simulink model "TP10_Examen_essuie_glaces_automatiques_simulink"  (R2022b)
settings: Solver=VariableStepAuto  StartTime=0.0  StopTime=inf  RelTol=1e-3
libraries: simulink x12
settings Model: Creator=HP  LastModifiedBy=HP

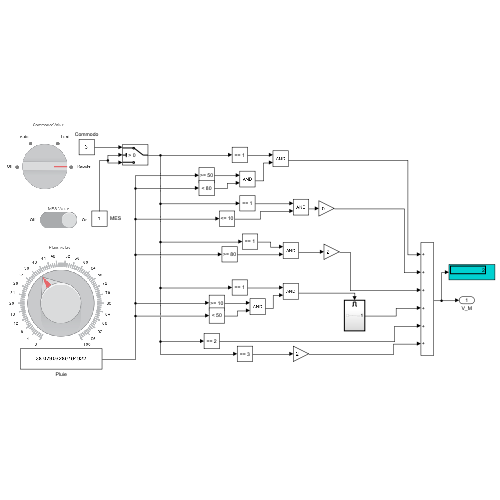
[thumbnail: Simulink's stored preview of the top-level diagram]
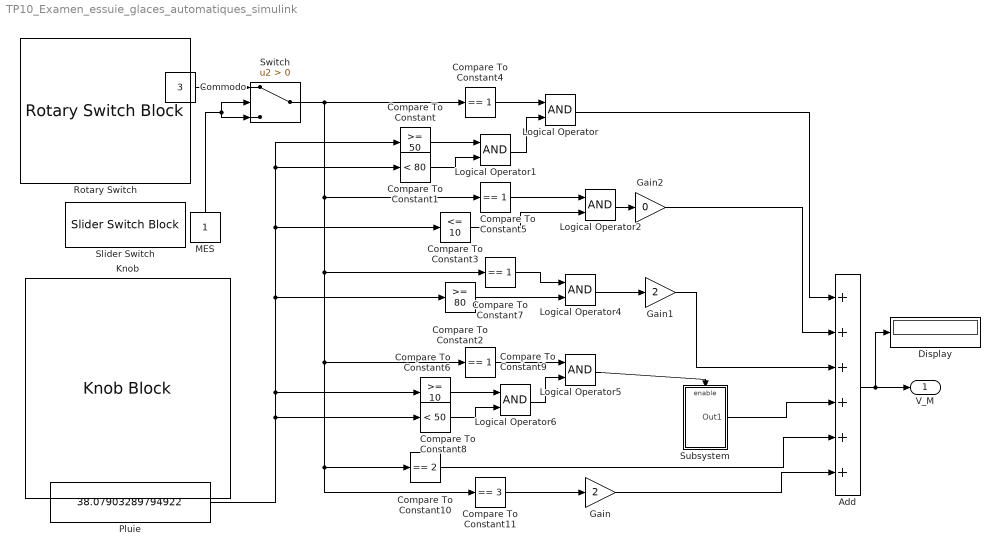
== system TP10_Examen_essuie_glaces_automatiques_simulink ==
  Add : Sum  Inputs=6
  Commodo : Constant  Value=3
  Compare To Constant : simulink/Logic and Bit Operations/Compare To Constant  relop=>=  const=50  OutDataTypeStr=boolean
  Compare To Constant1 : simulink/Logic and Bit Operations/Compare To Constant  relop=<  const=80  OutDataTypeStr=boolean
  Compare To Constant10 : simulink/Logic and Bit Operations/Compare To Constant  relop===  const=2  OutDataTypeStr=boolean
  Compare To Constant11 : simulink/Logic and Bit Operations/Compare To Constant  relop===  const=3  OutDataTypeStr=boolean
  Compare To Constant2 : simulink/Logic and Bit Operations/Compare To Constant  relop=>=  const=80  OutDataTypeStr=boolean
  Compare To Constant3 : simulink/Logic and Bit Operations/Compare To Constant  relop=<=  const=10  OutDataTypeStr=boolean
  Compare To Constant{4..5,7,9} (4 alike) : simulink/Logic and Bit Operations/Compare To Constant  relop===  const=1  OutDataTypeStr=boolean
  Compare To Constant6 : simulink/Logic and Bit Operations/Compare To Constant  relop=>=  const=10  OutDataTypeStr=boolean
  Compare To Constant8 : simulink/Logic and Bit Operations/Compare To Constant  relop=<  const=50  OutDataTypeStr=boolean
  Display : Display
  Gain : Gain  Gain=2
  Gain1 : Gain  Gain=2
  Gain2 : Gain  Gain=0
  Knob : KnobBlock
  Logical Operator{,1..2,4..6} (6 alike) : Logic  AllPortsSameDT=off  OutDataTypeStr=boolean
  MES : Constant
  Pluie : Constant  Value=38.07903289794922
  Rotary Switch : RotarySwitchBlock
      settings: Values={{'Off', 'Auto', 'Lent', 'Rapide'}, [0 1 2 3]}
  Slider Switch : SliderSwitchBlock
      settings: Values={{'Off', 'On'}, [0 1]}
  Subsystem : Subsystem
  Switch : Switch  Criteria=u2 > Threshold  SaturateOnIntegerOverflow=off  InputSameDT=off
  V_M : Outport
  wires:
  Commodo/1 -> Switch/1
  MES/1 -> Switch/2, Switch/3
  Compare To Constant/1 -> Logical Operator1/1
  Compare To Constant1/1 -> Logical Operator1/2
  Logical Operator1/1 -> Logical Operator/2
  Compare To Constant3/1 -> Logical Operator2/2
  Compare To Constant4/1 -> Logical Operator/1
  Compare To Constant5/1 -> Logical Operator2/1
  Switch/1 -> Compare To Constant5/1, Compare To Constant11/1, Compare To Constant10/1, Compare To Constant9/1, Compare To Constant7/1, Compare To Constant4/1
  Compare To Constant7/1 -> Logical Operator4/1
  Logical Operator4/1 -> Gain1/1
  Compare To Constant2/1 -> Logical Operator4/2
  Pluie/1 -> Compare To Constant3/1, Compare To Constant/1, Compare To Constant1/1, Compare To Constant2/1, Compare To Constant6/1, Compare To Constant8/1
  Compare To Constant9/1 -> Logical Operator5/1
  Logical Operator6/1 -> Logical Operator5/2
  Compare To Constant8/1 -> Logical Operator6/2
  Compare To Constant6/1 -> Logical Operator6/1
  Logical Operator5/1 -> Subsystem/Enable
  Compare To Constant10/1 -> Add/5
  Compare To Constant11/1 -> Gain/1
  Gain/1 -> Add/6
  Subsystem/1(Out1) -> Add/4
  Logical Operator/1 -> Add/1
  Logical Operator2/1 -> Gain2/1
  Add/1 -> V_M/1, Display/1
  Gain1/1 -> Add/3
  Gain2/1 -> Add/2

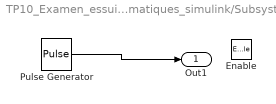
== system TP10_Examen_essuie_glaces_automatiques_simulink/Subsystem ==
  Enable : EnablePort
  Pulse Generator : DiscretePulseGenerator  PulseType=Time based  Period=4  PulseWidth=25
  Out1 : Outport
  wires:
  Pulse Generator/1 -> Out1/1
